simulink model "anjaneya_V9_fixed"  (R2025a)
settings: Solver=VariableStepAuto  StartTime=0.0  StopTime=100000  MaxStep=0.05  RelTol=1e-6
settings Model: Creator=kuppa  LastModifiedBy=saswat0907
settings DataIOCC: SaveFormat=StructureWithTime  ReturnWorkspaceOutputs=off

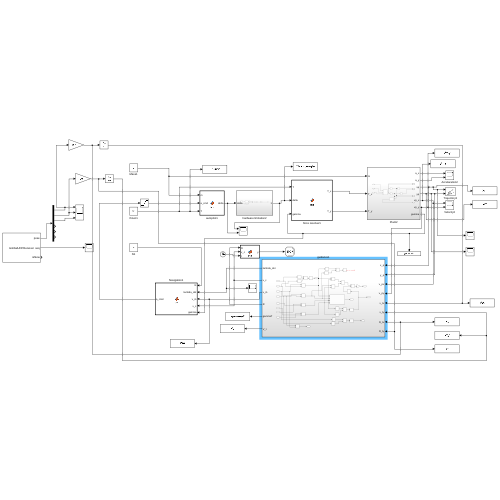
[thumbnail: Simulink's stored preview of the top-level diagram]
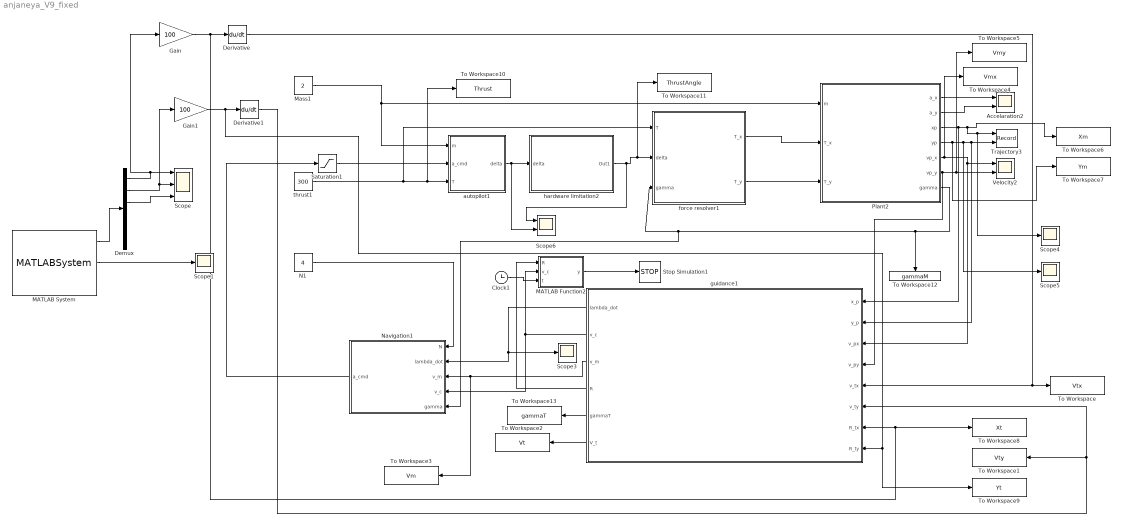
== system anjaneya_V9_fixed ==
  Accelaration2 : Scope  NumInputPorts=2
      settings: ActiveDisplayYMinimum=-670.09529615601855  ActiveDisplayYMaximum=430.47468331187889  DataLoggingVariableName=ScopeData6
  Clock1 : Clock
  Demux : Demux  Outputs=6
  Derivative : Derivative
  Derivative1 : Derivative
  Gain : Gain  Gain=100
  Gain1 : Gain  Gain=100
  MATLAB Function2 : MATLAB Function  TreatAsAtomicUnit=on
  MATLAB System : MATLABSystem  System=GimbalUDPReceiver  Port=25000  SimulateUsing=Interpreted execution
      mask Type: GimbalUDPReceiver
  Mass1 : Constant  Value=2
  N1 : Constant  Value=4
  Navigation1 : MATLAB Function  TreatAsAtomicUnit=on
  Plant2 : Subsystem
  Saturation1 : Saturate  UpperLimit=108  LowerLimit=-108
  Scope : Scope  NumInputPorts=3
      settings: ActiveDisplayYMinimum=-1.3912194659719609E-5  ActiveDisplayYMaximum=-7.1537397454231093E-7
  Scope{1,3..5} (4 alike) : Scope
      Scope3 settings: ActiveDisplayYMinimum=-0.71496170094090172  ActiveDisplayYMaximum=0.65598998004867615  DataLoggingVariableName=ScopeData7
      Scope4 settings: ActiveDisplayYMinimum=-25.430213641107127  ActiveDisplayYMaximum=35.257283778105105  DataLoggingVariableName=ScopeData8
      Scope5 settings: ActiveDisplayYMinimum=-57949.429144793568  ActiveDisplayYMaximum=306802.48338816618  DataLoggingVariableName=ScopeData9
  Scope6 : Scope  NumInputPorts=2
      settings: ActiveDisplayYMinimum=-0.11805254767904227  ActiveDisplayYMaximum=1.5944941621160178  DataLoggingVariableName=ScopeData5
  Stop Simulation1 : Stop
  To Workspace : ToWorkspace  VariableName=Vtx  SaveFormat=Timeseries  SampleTime=-1
  To Workspace1 : ToWorkspace  VariableName=Vty  SaveFormat=Timeseries  SampleTime=-1
  To Workspace10 : ToWorkspace  VariableName=Thrust  SaveFormat=Timeseries  SampleTime=-1
  To Workspace11 : ToWorkspace  VariableName=ThrustAngle  SaveFormat=Timeseries  SampleTime=-1
  To Workspace12 : ToWorkspace  VariableName=gammaM  SaveFormat=Timeseries  SampleTime=-1
  To Workspace13 : ToWorkspace  VariableName=gammaT  SaveFormat=Timeseries  SampleTime=-1
  To Workspace2 : ToWorkspace  VariableName=Vt  SaveFormat=Timeseries  SampleTime=-1
  To Workspace3 : ToWorkspace  VariableName=Vm  SaveFormat=Timeseries  SampleTime=-1
  To Workspace4 : ToWorkspace  VariableName=Vmx  SaveFormat=Timeseries  SampleTime=-1
  To Workspace5 : ToWorkspace  VariableName=Vmy  SaveFormat=Timeseries  SampleTime=-1
  To Workspace6 : ToWorkspace  VariableName=Xm  SaveFormat=Timeseries  SampleTime=-1
  To Workspace7 : ToWorkspace  VariableName=Ym  SaveFormat=Timeseries  SampleTime=-1
  To Workspace8 : ToWorkspace  VariableName=Xt  SaveFormat=Timeseries  SampleTime=-1
  To Workspace9 : ToWorkspace  VariableName=Yt  SaveFormat=Timeseries  SampleTime=-1
  Trajectory3 : Record  NumPorts=2.0  FileSettingsInternal="{\"entries\":[{\"content\":{\"excelSettings\":{\"content\":{},\"type\":\"Streamout.ExcelSettings\"},\"parquetSettings\":{\"content\":{},\"type\":\"Streamout.ParquetSettings\"}},\"type\":\"Streamout.FileSettingStorage\",\"uuid\":\"\"}],\"packageUris\":[\"http:\\/\\/schema.mathworks.com\\/mf0\\/streamout_blocks\\/R2020a\"],\"version\":\"1.0\"}"  FrameSettings=[0, 0]  Layout=[1 1]  SignalsInternal="{\"entries\":[{\"content\":{\"signals\":[{\"content\":{\"blockPath\":[],\"dimensions\":[1],\"domain\":\"\",\"lineColor\":\"#64d413\",\"lineWidth\":2,\"port\":1,\"signalID\":1,\"signalName\":\"Plant2:3\"},\"type\":\"RecordBlkView.Signal\",\"uuid\":\"\"},{\"content\":{\"blockPath\":[],\"dimensions\":[1],\"domain\":\"\",\"lineColor\":\"#ff13a6\",\"lineWidth\":2,\"port\":2,\"signalID\":2,\"signalName\":\"Plant2:4\"},\"type\":\"RecordBlkView.Signal\",\"uuid\":\"\"}]},\"type\":\"RecordBlkView.InputSignals\",\"uuid\":\"\"}],\"packageUris\":[\"http:\\/\\/schema.mathworks.com\\/mf0\\/streamout_blocks\\/R2020a\"],\"version\":\"1.0\"}"  VisualizationBindings="{\"xyplotplugin\":{\"info\":[{\"series\":[],\"subplotID\":1}]}}"  CompatibilityTag=XY
  Velocity2 : Scope  NumInputPorts=2
      settings: ActiveDisplayYMinimum=-149.61714228527322  ActiveDisplayYMaximum=359.76787547365052  DataLoggingVariableName=ScopeData10
  autopilot1 : MATLAB Function  TreatAsAtomicUnit=on
  force resolver1 : MATLAB Function  TreatAsAtomicUnit=on
  guidance1 : Subsystem
  hardware limitation2 : Subsystem
  thrust1 : Constant  Value=300
  wires:
  Saturation1/1 -> autopilot1/2(a_cmd)
  Plant2/4(yp) -> To Workspace7/1, Scope5/1, guidance1/2(y_p), Trajectory3/2
  guidance1/5(gammaT) -> To Workspace13/1
  Plant2/5(vp_x) -> To Workspace4/1, guidance1/3(v_px), Velocity2/1
  Navigation1/1(a_cmd) -> Saturation1/1
  guidance1/1(lambda_dot) -> Navigation1/2(lambda_dot), Scope3/1
  Plant2/2(a_y) -> Accelaration2/2
  force resolver1/2(T_y) -> Plant2/3(T_y)
  Clock1/1 -> MATLAB Function2/3(t)
  Plant2/6(vp_y) -> guidance1/4(v_py), To Workspace5/1, Velocity2/2
  MATLAB Function2/1(y) -> Stop Simulation1/1
  thrust1/1 -> To Workspace10/1, autopilot1/3(T), force resolver1/1(T)
  guidance1/3(v_m) -> To Workspace3/1, Navigation1/3(v_m)
  guidance1/2(v_c) -> MATLAB Function2/2(v_c), Navigation1/4(v_c)
  Derivative/1 -> To Workspace/1, guidance1/5(v_tx)
  Plant2/1(a_x) -> Accelaration2/1
  N1/1 -> Navigation1/1(N)
  Plant2/3(xp) -> To Workspace6/1, Scope4/1, Trajectory3/1, guidance1/1(x_p)
  force resolver1/1(T_x) -> Plant2/2(T_x)
  Plant2/7(gamma) -> Navigation1/5(gamma), force resolver1/3(gamma), To Workspace12/1
  Mass1/1 -> autopilot1/1(m), Plant2/1(m)
  guidance1/4(R) -> MATLAB Function2/1(R)
  autopilot1/1(delta) -> hardware limitation2/1(delta), Scope6/2
  Derivative1/1 -> guidance1/6(v_ty), To Workspace1/1
  hardware limitation2/1(Out1) -> Scope6/1, To Workspace11/1, force resolver1/2(delta)
  guidance1/6(V_t) -> To Workspace2/1
  MATLAB System/1 -> Demux/1
  Demux/1 -> Scope/1, Gain/1
  Demux/2 -> Gain1/1, Scope/2
  Demux/3 -> Scope/3
  MATLAB System/2 -> Scope1/1
  Gain/1 -> guidance1/7(R_tx), To Workspace8/1, Derivative/1
  Gain1/1 -> To Workspace9/1, guidance1/8(R_ty), Derivative1/1

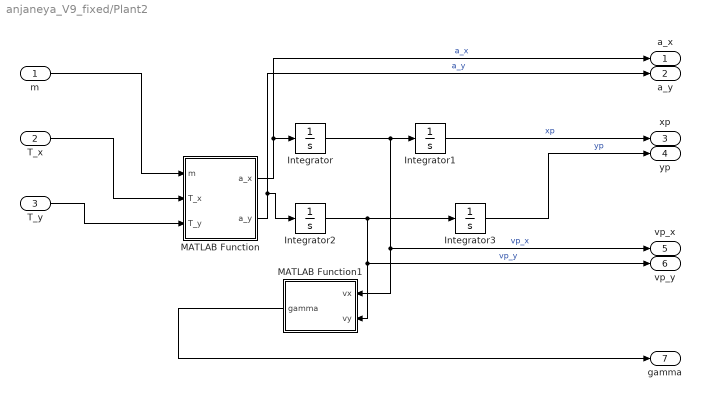
== system anjaneya_V9_fixed/Plant2 ==
  m : Inport
  T_x : Inport  Port=2
  T_y : Inport  Port=3
  Integrator : Integrator  InitialCondition=0.5
  Integrator1 : Integrator
  Integrator2 : Integrator  InitialCondition=0.5
  Integrator3 : Integrator
  MATLAB Function : MATLAB Function  TreatAsAtomicUnit=on
  MATLAB Function1 : MATLAB Function  TreatAsAtomicUnit=on
  a_x : Outport
  a_y : Outport  Port=2
  xp : Outport  Port=3
  yp : Outport  Port=4
  vp_x : Outport  Port=5
  vp_y : Outport  Port=6
  gamma : Outport  Port=7
  wires:
  m/1 -> MATLAB Function/1(m)
  MATLAB Function/2(a_y) -> Integrator2/1, a_y/1  "a_y"
  Integrator/1 -> Integrator1/1, vp_x/1, MATLAB Function1/1(vx)  "vp_x"
  Integrator2/1 -> Integrator3/1, vp_y/1, MATLAB Function1/2(vy)  "vp_y"
  T_x/1 -> MATLAB Function/2(T_x)
  T_y/1 -> MATLAB Function/3(T_y)
  MATLAB Function/1(a_x) -> Integrator/1, a_x/1  "a_x"
  Integrator3/1 -> yp/1  "yp"
  Integrator1/1 -> xp/1  "xp"
  MATLAB Function1/1(gamma) -> gamma/1

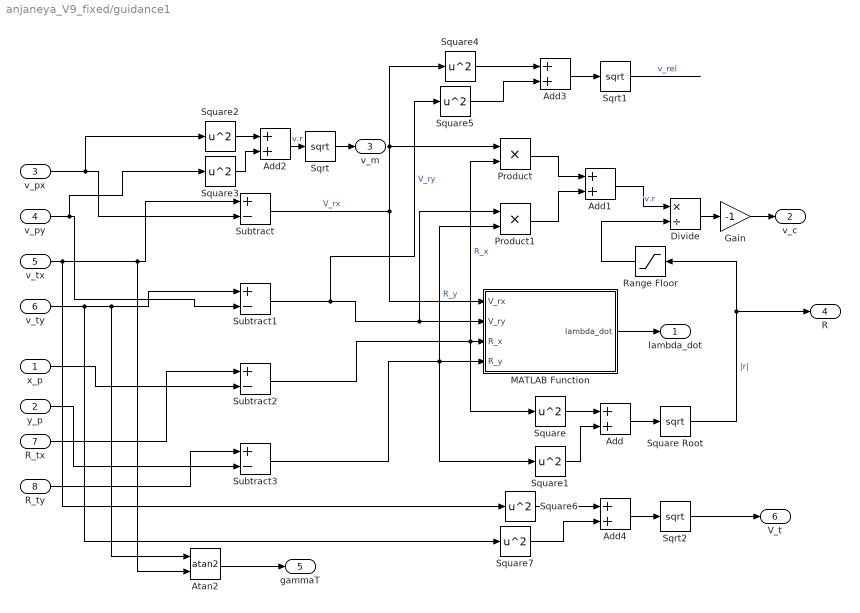
== system anjaneya_V9_fixed/guidance1 ==
  x_p : Inport
  y_p : Inport  Port=2
  v_px : Inport  Port=3
  v_py : Inport  Port=4
  v_tx : Inport  Port=5
  v_ty : Inport  Port=6
  R_tx : Inport  Port=7
  R_ty : Inport  Port=8
  Add{,1..4} (5 alike) : Sum
  Atan2 : Trigonometry  Operator=atan2
  Divide : Product  Inputs=*/
  Gain : Gain  Gain=-1
  MATLAB Function : MATLAB Function  TreatAsAtomicUnit=on
  Product : Product
  Product1 : Product
  Range Floor : Saturate  UpperLimit=Inf  LowerLimit=1e-3
  Sqrt : Sqrt
  Sqrt1 : Sqrt
  Sqrt2 : Sqrt
  Square{,1..7} (8 alike) : Math  Operator=square
  Square Root : Sqrt
  Subtract{,1..3} (4 alike) : Sum  Inputs=+-
  lambda_dot : Outport
  v_c : Outport  Port=2
  v_m : Outport  Port=3
  R : Outport  Port=4
  gammaT : Outport  Port=5
  V_t : Outport  Port=6
  wires:
  x_p/1 -> Subtract2/2
  v_tx/1 -> Square6/1, Atan2/2, Subtract/1
  v_px/1 -> Square2/1, Subtract/2
  Subtract/1 -> Square4/1, Product/1, MATLAB Function/1(V_rx)  "V_rx"
  v_ty/1 -> Square7/1, Atan2/1, Subtract1/1
  v_py/1 -> Square3/1, Subtract1/2
  Subtract1/1 -> Square5/1, MATLAB Function/2(V_ry), Product1/1  "V_ry"
  R_tx/1 -> Subtract2/1
  R_ty/1 -> Subtract3/1
  y_p/1 -> Subtract3/2
  Subtract2/1 -> Square/1, MATLAB Function/3(R_x), Product/2  "R_x"
  Subtract3/1 -> MATLAB Function/4(R_y), Product1/2, Square1/1  "R_y"
  MATLAB Function/1(lambda_dot) -> lambda_dot/1
  Square/1 -> Add/1
  Square1/1 -> Add/2
  Add/1 -> Square Root/1
  Square Root/1 -> Range Floor/1, R/1  "|r|"
  Range Floor/1 -> Divide/2
  Product/1 -> Add1/1
  Product1/1 -> Add1/2
  Add1/1 -> Divide/1  "v.r"
  Divide/1 -> Gain/1
  Gain/1 -> v_c/1
  Square2/1 -> Add2/1
  Square3/1 -> Add2/2
  Add2/1 -> Sqrt/1  "v.r"
  Sqrt/1 -> v_m/1
  Atan2/1 -> gammaT/1
  Square4/1 -> Add3/1
  Square5/1 -> Add3/2
  Add3/1 -> Sqrt1/1
  Sqrt1/1 -> ?  "v_rel"
  Add4/1 -> Sqrt2/1
  Square7/1 -> Add4/2
  Sqrt2/1 -> V_t/1
  Square6/1 -> Add4/1

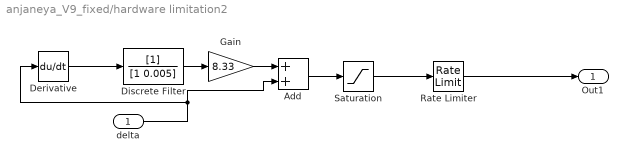
== system anjaneya_V9_fixed/hardware limitation2 ==
  delta : Inport
  Add : Sum
  Derivative : Derivative
  Discrete Filter : DiscreteFilter  Denominator=[1 0.005]
  Gain : Gain  Gain=8.33
  Rate Limiter : RateLimiter  RisingSlewLimit=0.523  FallingSlewLimit=-0.523  SampleTimeMode=inherited
  Saturation : Saturate  UpperLimit=0.72  LowerLimit=-0.72
  Out1 : Outport
  wires:
  Saturation/1 -> Rate Limiter/1
  Rate Limiter/1 -> Out1/1
  delta/1 -> Derivative/1, Add/2
  Derivative/1 -> Discrete Filter/1
  Discrete Filter/1 -> Gain/1
  Gain/1 -> Add/1
  Add/1 -> Saturation/1

== matlab function anjaneya_V9_fixed/MATLAB Function2 ==
  data: R input; v_c input; y output; t input
function y = fcn(R, v_c, t)
    if t > 0.05 && (R < 0.5 || v_c <= 0) && t<100000
        y = 1;
    else
        y = 0;
    end
end

== matlab function anjaneya_V9_fixed/Navigation1 ==
  data: N input; a_cmd output; lambda_dot input; v_m input; v_c input; gamma input
function a_cmd = fcn(N, lambda_dot, v_m, v_c, gamma)
    g = 9.81;

    if v_c > 0 
        a_guide = N * v_m * lambda_dot;
    else
        a_guide = 0;
    end
    
    a_grav = g * cos(gamma);

    a_cmd = a_guide + a_grav;
end

== matlab function anjaneya_V9_fixed/Plant2/MATLAB Function ==
  data: m input; T_x input; T_y input; a_x output; a_y output
function [a_x,a_y]= fcn(m, T_x, T_y)

g = 9.81;
a_x = (T_x)/m;
a_y = ((T_y)/m -g);

== matlab function anjaneya_V9_fixed/Plant2/MATLAB Function1 ==
  data: vx input; gamma output; vy input
function gamma = fcn(vx, vy)

gamma = atan2(vy,vx);

== matlab function anjaneya_V9_fixed/autopilot1 ==
  data: m input; a_cmd input; delta output; T input
function delta = fcn(m, a_cmd, T)
    s = m * a_cmd / T;
    s = max(min(s, 0.99), -0.99);
    delta = asin(s);
end

== matlab function anjaneya_V9_fixed/force resolver1 ==
  data: T input; delta input; gamma input; T_x output; T_y output
function [T_x , T_y] = fcn(T , delta , gamma)

theta_T = delta + gamma;
T_x = T*cos(theta_T);
T_y = T*sin(theta_T);

== matlab function anjaneya_V9_fixed/guidance1/MATLAB Function ==
  data: V_rx input; lambda_dot output; V_ry input; R_x input; R_y input
function lambda_dot = fcn(V_rx, V_ry, R_x, R_y)

R_square = R_x*R_x + R_y*R_y;
lambda_dot = (R_x*V_ry - R_y*V_rx )/R_square ;
